simulink model "emso1"  (Simulink 7.1)
settings: Solver=VariableStepDiscrete  StartTime=0.0  StopTime=360  RelTol=1e-3
settings Model: Creator=lades  LastModifiedBy=lades
settings DataIOCC: ExternalInput=Az

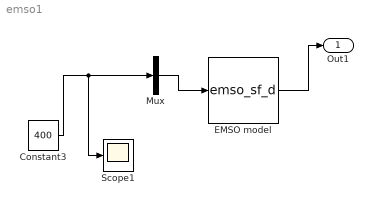
== system emso1 ==
  Constant3 : Constant  Value=400  OutDataType=sfix(16)  OutScaling=2^0
  EMSO model : S-Function  FunctionName=emso_sf_d  Parameters='Acetic.ems',1,1,1  EnableBusSupport=off
  Mux : Mux  Inputs=1
  Scope1 : Scope
      settings: TimeRange=2  YMin=4.008258966500001  YMax=4.008258969500001
  Out1 : Outport  OutDataType=sfix(16)  OutScaling=2^0
  wires:
  EMSO model/1 -> Out1/1
  Mux/1 -> EMSO model/1
  Constant3/1 -> Mux/1, Scope1/1
